simulink model "MPC_RobotM"  (R2026b)
settings: Solver=ode1  StartTime=0.01  StopTime=360  FixedStep=0.02
undefined symbols (not defined in the file or in its folder): K_c
libraries: vrlib x2, slpidlib x2
settings Model: Creator=Tom  LastModifiedBy=Tom

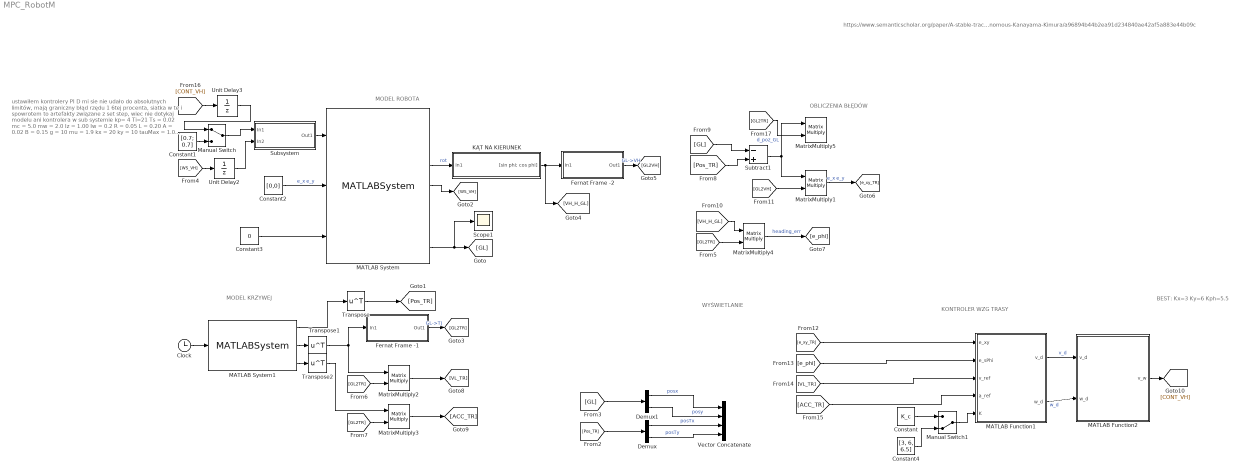
== system MPC_RobotM ==
  note: KONTROLER WZG TRASY
  note: OBLICZENIA BŁĘDÓW
  note: MODEL KRZYWEJ
  note: MODEL ROBOTA
  note: WYŚWIETLANIE
  note: https://www.semanticscholar.org/paper/A-stable-tracking-control-method-for-an-autonomous-Kanayama-Kimura/a96894b44b2ea91d234840ae42af5a883e44b09c
  note: ustawiłem kontrolery PI D mi sie nie udało do absolutnych limitów, mają graniczny błąd rzędu 1 6tej procenta, siatka w te i spowrotem to artefakty związane z set step, wiec nie dotykaj modelu ani kontrolera w sub systemie kp= 4 Ti=21
      | Ts = 0.02
      | mc = 5.0
      | mw = 2.0
      | Iz = 1.00
      | Iw = 0.2
      | R = 0.05
      | L = 0.20
      | A = 0.02
      | B = 0.15
      | g = 10
      | mu = 1.9
      | kx = 20
      | ky = 10
      | tauMax = 1.0
      | wMax = 20
      | tauF = 0.05
  note: BEST:
      | Kx=3
      | Ky=6
      | Kph=5.5
  Clock : Clock
  Constant : Constant  Value=K_c
  Constant1 : Constant  Value=[0.7; 0.7]
  Constant2 : Constant  Value=[0,0]  SampleTime=-1
  Constant3 : Constant  Value=0  SampleTime=-1
  Constant4 : Constant  Value=[3, 6, 6.5]
  Demux : Demux  Outputs=2
  Demux1 : Demux  Outputs=2
  Fernat Frame -1 : Subsystem
  Fernat Frame -2 : Subsystem
  KĄT NA KIERUNEK : Subsystem
  MATLAB Function1 : MATLAB Function  TreatAsAtomicUnit=on
  MATLAB Function2 : MATLAB Function  TreatAsAtomicUnit=on
  MATLAB System : MATLABSystem  System=RobotMobilny  Ts=0.02  mc=5  mw=2  Iz=1.00  Iw=0.2  R=0.05  L=0.20  A=0.02  B=0.15  g=10  mu=1.9  kx=20  ky=10  tauMax=1.0  wMax=20  tauF=0.05  SimulateUsing=Code generation
  MATLAB System1 : MATLABSystem  System=CubicBCurve2System  ControlPoints=[0, 10, 20, 30; 0, 10, 0, 10]  alpha=0.5  beta=0.4  startSpeed=0  endSpeed=0  SegmentTimes="[120\t120\t120]"  SimulateUsing=Interpreted execution
  Manual Switch : ManualSwitch
  Manual Switch1 : ManualSwitch  CurrentSetting=0
  MatrixMultiply{1..5} (5 alike) : Product  Multiplication=Matrix(*)
  Scope1 : Scope
      settings: ActiveDisplayYMinimum=-1  ActiveDisplayYMaximum=1  DataLoggingVariableName=ScopeData2
  Subsystem : Subsystem
  Subtract1 : Sum  Inputs=-+
  Transpose : Math  Operator=transpose
  Transpose1 : Math  Operator=transpose
  Transpose2 : Math  Operator=transpose
  Unit Delay2 : UnitDelay  SampleTime=-1
  Unit Delay3 : UnitDelay  SampleTime=-1
  Vector Concatenate : Concatenate  NumInputs=4
  wires:
  Constant3/1 -> MATLAB System/3
  MATLAB System/4 -> [WS_VH]
  Subsystem/1(Out1) -> MATLAB System/1
  MATLAB System1/1 -> Transpose/1
  MATLAB System1/2 -> Transpose1/1
  MATLAB System1/3 -> Transpose2/1
  MATLAB Function1/1(v_d) -> MATLAB Function2/1(v_d)  "v_d"
  MATLAB Function1/2(w_d) -> MATLAB Function2/2(w_d)  "w_d"
  [Pos_TR] -> Demux/1
  [GL] -> Demux1/1
  KĄT NA KIERUNEK/1("[sin phi; cos phi]") -> Fernat Frame -2/1(In1), [VH_H_GL]
  MATLAB System/3 -> KĄT NA KIERUNEK/1(In1)  "rot"
  [WS_VH] -> Unit Delay2/1
  Unit Delay2/1 -> Subsystem/2(In2)
  Fernat Frame -1/1(Out1) -> [GL2TR]  "GL->TJ"
  [GL2TR] -> MatrixMultiply4/2
  [GL2TR] -> MatrixMultiply2/2
  [GL2TR] -> MatrixMultiply3/2
  Subtract1/1 -> MatrixMultiply1/1, MatrixMultiply5/1  "d_poz_GL"
  [VH_H_GL] -> MatrixMultiply4/1
  Fernat Frame -2/1(Out1) -> [GL2VH]  "GL->VH"
  [GL2VH] -> MatrixMultiply1/2
  MatrixMultiply1/1 -> [e_xy_TR]  "e_x e_y"
  [e_xy_TR] -> MATLAB Function1/1(e_xy)
  MatrixMultiply4/1 -> [e_phi]  "heading_err"
  [e_phi] -> MATLAB Function1/2(e_sPhi)
  MatrixMultiply2/1 -> [VL_TR]
  [VL_TR] -> MATLAB Function1/3(v_ref)
  MatrixMultiply3/1 -> [ACC_TR]
  [ACC_TR] -> MATLAB Function1/4(a_ref)
  MATLAB Function2/1(v_w) -> [CONT_VH]
  [CONT_VH] -> Unit Delay3/1
  Constant2/1 -> MATLAB System/2  "e_x e_y"
  MATLAB System/7 -> Scope1/1, [GL]
  Unit Delay3/1 -> Manual Switch/1
  Manual Switch/1 -> Subsystem/1(In1)
  Constant1/1 -> Manual Switch/2
  Transpose/1 -> [Pos_TR]
  Transpose1/1 -> Fernat Frame -1/1(In1), MatrixMultiply2/1
  Transpose2/1 -> MatrixMultiply3/1
  [GL] -> Subtract1/1
  [Pos_TR] -> Subtract1/2
  Demux/2 -> Vector Concatenate/4  "posTy"
  Demux/1 -> Vector Concatenate/3  "posTx"
  Demux1/2 -> Vector Concatenate/2  "posy"
  Demux1/1 -> Vector Concatenate/1  "posx"
  [GL2TR] -> MatrixMultiply5/2
  Clock/1 -> MATLAB System1/1
  Constant4/1 -> Manual Switch1/2
  Manual Switch1/1 -> MATLAB Function1/5(K)
  Constant/1 -> Manual Switch1/1

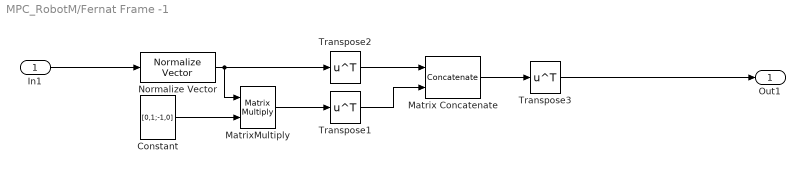
== system MPC_RobotM/Fernat Frame -1 ==
  In1 : Inport
  Constant : Constant  Value=[0,1;-1,0]
  Matrix Concatenate : Concatenate  Mode=Multidimensional array  ConcatenateDimension=2
  MatrixMultiply : Product  Multiplication=Matrix(*)
  Normalize Vector : vrlib/Utilities/Normalize Vector  maxzero=0
  Transpose1 : Math  Operator=transpose
  Transpose2 : Math  Operator=transpose
  Transpose3 : Math  Operator=transpose
  Out1 : Outport
  wires:
  Constant/1 -> MatrixMultiply/2
  MatrixMultiply/1 -> Transpose1/1
  Normalize Vector/1 -> MatrixMultiply/1, Transpose2/1
  Matrix Concatenate/1 -> Transpose3/1
  Transpose1/1 -> Matrix Concatenate/2
  Transpose2/1 -> Matrix Concatenate/1
  Transpose3/1 -> Out1/1
  In1/1 -> Normalize Vector/1

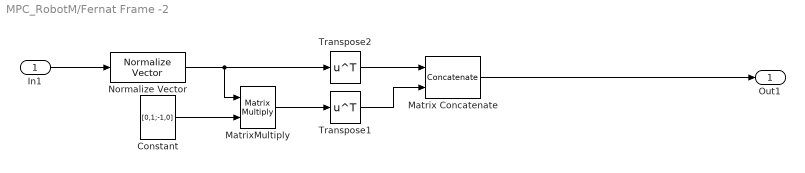
== system MPC_RobotM/Fernat Frame -2 ==
  In1 : Inport
  Constant : Constant  Value=[0,1;-1,0]
  Matrix Concatenate : Concatenate  Mode=Multidimensional array  ConcatenateDimension=2
  MatrixMultiply : Product  Multiplication=Matrix(*)
  Normalize Vector : vrlib/Utilities/Normalize Vector  maxzero=0
  Transpose1 : Math  Operator=transpose
  Transpose2 : Math  Operator=transpose
  Out1 : Outport
  wires:
  Constant/1 -> MatrixMultiply/2
  MatrixMultiply/1 -> Transpose1/1
  Normalize Vector/1 -> MatrixMultiply/1, Transpose2/1
  In1/1 -> Normalize Vector/1
  Matrix Concatenate/1 -> Out1/1
  Transpose1/1 -> Matrix Concatenate/2
  Transpose2/1 -> Matrix Concatenate/1

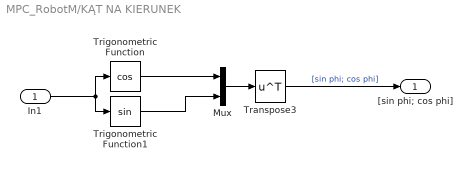
== system MPC_RobotM/KĄT NA KIERUNEK ==
  In1 : Inport
  Mux : Mux  Inputs=2
  Transpose3 : Math  Operator=transpose
  Trigonometric Function : Trigonometry  Operator=cos
  Trigonometric Function1 : Trigonometry
  "[sin phi; cos phi]" : Outport
  wires:
  Trigonometric Function1/1 -> Mux/2
  Trigonometric Function/1 -> Mux/1
  Mux/1 -> Transpose3/1
  In1/1 -> Trigonometric Function1/1, Trigonometric Function/1
  Transpose3/1 -> "[sin phi; cos phi]"/1  "[sin phi; cos phi]"

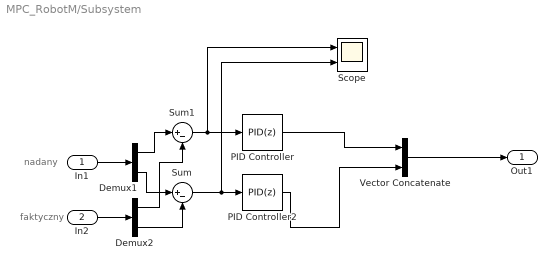
== system MPC_RobotM/Subsystem ==
  note: faktyczny
  note: nadany
  In1 : Inport
  In2 : Inport  Port=2
  Demux1 : Demux  Outputs=2
  Demux2 : Demux  Outputs=2
  PID Controller : slpidlib/PID Controller  Controller=PID  Form=Parallel  TimeDomain=Discrete-time  UseExternalTs=off  SampleTime=-1  IntegratorMethod=Forward Euler  FilterMethod=Forward Euler  ControllerParametersSource=internal  P=4  I=21  UseKiTs=off  D=0  UseExternalDerivativeSource=off  N=10  UseFilter=on  TunerSelectOption=Transfer Function Based (PID Tuner App)  InitialConditionSource=internal  InitialConditionForIntegrator=0  InitialConditionForFilter=0  DifferentiatorICPrevScaledInput=0  ExternalReset=none  TrackingMode=off  Kt=1  LimitOutput=on  SatLimitsSource=internal  UpperSaturationLimit=1  LowerSaturationLimit=-1  LinearizeAsGain=on  AntiWindupMode=clamping  Kb=1  LimitIntegrator=off  UpperIntegratorSaturationLimit=inf  LowerIntegratorSaturationLimit=-inf  POutMin=[]  POutMax=[]  IOutMin=[]  IOutMax=[]  DOutMin=[]  DOutMax=[]  NOutMin=[]  NOutMax=[]  SumOutMin=[]  SumOutMax=[]  SaturationOutMin=[]  SaturationOutMax=[]  PParamMin=[]  PParamMax=[]  IParamMin=[]  IParamMax=[]  DParamMin=[]  DParamMax=[]  NParamMin=[]  NParamMax=[]  KbParamMin=[]  KbParamMax=[]  KtParamMin=[]  KtParamMax=[]  KbOutMin=[]  KbOutMax=[]  KtOutMin=[]  KtOutMax=[]  IntegratorOutMin=[]  IntegratorOutMax=[]  FilterOutMin=[]  FilterOutMax=[]  SumI1OutMin=[]  SumI1OutMax=[]  SumI2OutMin=[]  SumI2OutMax=[]  SumI3OutMin=[]  SumI3OutMax=[]  SumI4OutMin=[]  SumI4OutMax=[]  SumDOutMin=[]  SumDOutMax=[]  DifferentiatorOutMin=[]  DifferentiatorOutMax=[]  FilterDiffOutCoefMin=[]  FilterDiffOutCoefMax=[]  ReciprocalOutMin=[]  ReciprocalOutMax=[]  SumDenOutMin=[]  SumDenOutMax=[]  SumNumOutMin=[]  SumNumOutMax=[]  DivideOutMin=[]  DivideOutMax=[]  UdiffTsProdOutMin=[]  UdiffTsProdOutMax=[]  NTsProdOutMin=[]  NTsProdOutMax=[]  UintegralTsProdOutMin=[]  UintegralTsProdOutMax=[]  UngainTsProdOutMin=[]  UngainTsProdOutMax=[]  ClampingZeroOutDataTypeStr=Inherit: Inherit via back propagation  ClampingZeroOutMin=[]  ClampingZeroOutMax=[]  FilterDenConstantOutDataTypeStr=Inherit: Inherit via back propagation  FilterDenConstantOutMin=[]  FilterDenConstantOutMax=[]  PCopyOutDataTypeStr=Inherit: Inherit via back propagation  PCopyOutMin=[]  PCopyOutMax=[]  NCopyOutDataTypeStr=Inherit: Inherit via back propagation  NCopyOutMin=[]  NCopyOutMax=[]  IntegratorContinuousStateAttributes=''  IntegratorStateMustResolveToSignalObject=off  IntegratorRTWStateStorageClass=Auto  FilterContinuousStateAttributes=''  FilterStateMustResolveToSignalObject=off  FilterRTWStateStorageClass=Auto  ParallelPVariant=InternalParameters  IdealPVariant=Disabled  IVariant=InternalParameters  DVariant=InternalParameters  IntegratorVariant=Discrete  SatVariant=Enabled  AWVariant=DiscClampingParallel  PCopyVariant=Disabled  TRVariant=Disabled  FdbkBlocksVariant=Forward  IdealPFdbkVariant=Disabled  SatFdbkVariant=Disabled  DerivativeFilterVariant=ForwardEulerFilter  NVariant=InternalParameters  NCopyVariant=Disabled  FilterICVariant=InternalICsFilter  IntegratorICVariant=InternalICs  ExternalResetVariant=Disabled  TRSumVariant=Passthrough  SumFdbkVariant=Disabled  SumVariant=Sum_PID  TsampFilterVariant=InternalTs  TsampNgainVariant=Passthrough  TsampIntegralVariant=Disabled_SignalSpec  ExternalSaturationOutDataTypeStr=Inherit: Same as second input  DerivativeSourceVariant=ErrorSignal  PreIntVariant=InternalPreInt
  PID Controller2 : slpidlib/PID Controller  Controller=PID  Form=Parallel  TimeDomain=Discrete-time  UseExternalTs=off  SampleTime=-1  IntegratorMethod=Forward Euler  FilterMethod=Forward Euler  ControllerParametersSource=internal  P=4  I=21  UseKiTs=off  D=0  UseExternalDerivativeSource=off  N=10  UseFilter=on  TunerSelectOption=Transfer Function Based (PID Tuner App)  InitialConditionSource=internal  InitialConditionForIntegrator=0  InitialConditionForFilter=0  DifferentiatorICPrevScaledInput=0  ExternalReset=none  TrackingMode=off  Kt=1  LimitOutput=on  SatLimitsSource=internal  UpperSaturationLimit=1  LowerSaturationLimit=-1  LinearizeAsGain=on  AntiWindupMode=clamping  Kb=1  LimitIntegrator=off  UpperIntegratorSaturationLimit=inf  LowerIntegratorSaturationLimit=-inf  POutMin=[]  POutMax=[]  IOutMin=[]  IOutMax=[]  DOutMin=[]  DOutMax=[]  NOutMin=[]  NOutMax=[]  SumOutMin=[]  SumOutMax=[]  SaturationOutMin=[]  SaturationOutMax=[]  PParamMin=[]  PParamMax=[]  IParamMin=[]  IParamMax=[]  DParamMin=[]  DParamMax=[]  NParamMin=[]  NParamMax=[]  KbParamMin=[]  KbParamMax=[]  KtParamMin=[]  KtParamMax=[]  KbOutMin=[]  KbOutMax=[]  KtOutMin=[]  KtOutMax=[]  IntegratorOutMin=[]  IntegratorOutMax=[]  FilterOutMin=[]  FilterOutMax=[]  SumI1OutMin=[]  SumI1OutMax=[]  SumI2OutMin=[]  SumI2OutMax=[]  SumI3OutMin=[]  SumI3OutMax=[]  SumI4OutMin=[]  SumI4OutMax=[]  SumDOutMin=[]  SumDOutMax=[]  DifferentiatorOutMin=[]  DifferentiatorOutMax=[]  FilterDiffOutCoefMin=[]  FilterDiffOutCoefMax=[]  ReciprocalOutMin=[]  ReciprocalOutMax=[]  SumDenOutMin=[]  SumDenOutMax=[]  SumNumOutMin=[]  SumNumOutMax=[]  DivideOutMin=[]  DivideOutMax=[]  UdiffTsProdOutMin=[]  UdiffTsProdOutMax=[]  NTsProdOutMin=[]  NTsProdOutMax=[]  UintegralTsProdOutMin=[]  UintegralTsProdOutMax=[]  UngainTsProdOutMin=[]  UngainTsProdOutMax=[]  ClampingZeroOutDataTypeStr=Inherit: Inherit via back propagation  ClampingZeroOutMin=[]  ClampingZeroOutMax=[]  FilterDenConstantOutDataTypeStr=Inherit: Inherit via back propagation  FilterDenConstantOutMin=[]  FilterDenConstantOutMax=[]  PCopyOutDataTypeStr=Inherit: Inherit via back propagation  PCopyOutMin=[]  PCopyOutMax=[]  NCopyOutDataTypeStr=Inherit: Inherit via back propagation  NCopyOutMin=[]  NCopyOutMax=[]  IntegratorContinuousStateAttributes=''  IntegratorStateMustResolveToSignalObject=off  IntegratorRTWStateStorageClass=Auto  FilterContinuousStateAttributes=''  FilterStateMustResolveToSignalObject=off  FilterRTWStateStorageClass=Auto  ParallelPVariant=InternalParameters  IdealPVariant=Disabled  IVariant=InternalParameters  DVariant=InternalParameters  IntegratorVariant=Discrete  SatVariant=Enabled  AWVariant=DiscClampingParallel  PCopyVariant=Disabled  TRVariant=Disabled  FdbkBlocksVariant=Forward  IdealPFdbkVariant=Disabled  SatFdbkVariant=Disabled  DerivativeFilterVariant=ForwardEulerFilter  NVariant=InternalParameters  NCopyVariant=Disabled  FilterICVariant=InternalICsFilter  IntegratorICVariant=InternalICs  ExternalResetVariant=Disabled  TRSumVariant=Passthrough  SumFdbkVariant=Disabled  SumVariant=Sum_PID  TsampFilterVariant=InternalTs  TsampNgainVariant=Passthrough  TsampIntegralVariant=Disabled_SignalSpec  ExternalSaturationOutDataTypeStr=Inherit: Same as second input  DerivativeSourceVariant=ErrorSignal  PreIntVariant=InternalPreInt
  Scope : Scope  NumInputPorts=2
      settings: ActiveDisplayYMinimum=-0.019248045487536222  ActiveDisplayYMaximum=0.016415708171777878
  Sum : Sum  Inputs=|+-
  Sum1 : Sum  Inputs=|+-
  Vector Concatenate : Concatenate
  Out1 : Outport
  wires:
  Vector Concatenate/1 -> Out1/1
  PID Controller2/1 -> Vector Concatenate/2
  In1/1 -> Demux1/1
  In2/1 -> Demux2/1
  Demux1/2 -> Sum/1
  Demux2/2 -> Sum/2
  Demux1/1 -> Sum1/1
  Demux2/1 -> Sum1/2
  Sum1/1 -> Scope/1, PID Controller/1
  Sum/1 -> Scope/2, PID Controller2/1
  PID Controller/1 -> Vector Concatenate/1

== matlab function MPC_RobotM/MATLAB Function1 ==
  data: e_xy input; v_d output; e_sPhi input; v_ref input; a_ref input; w_d output; K input
function [v_d, w_d] = kanayama(e_xy, e_sPhi, v_ref, a_ref, K)
kx = K(1); ky = K(2); kth = K(3);
eps_v = 1e-2;
v_r = v_ref(2);
w_r = a_ref(1) * v_r / (v_r^2 + eps_v^2);
%v_d = v_r * e_sPhi(2) + kx * e_xy(1);
v_d = max(v_r * e_sPhi(2) + kx * e_xy(1), 0);
w_d = w_r + v_r * (ky * e_xy(2) + kth * e_sPhi(1));
end

== matlab function MPC_RobotM/MATLAB Function2 ==
  data: v_d input; v_w output; w_d input
function v_w = Pred_LP(v_d, w_d)
L = 0.2;
v_w = [v_d - w_d * L/2;
    v_d + w_d * L/2];
end
